simulink library "flightgear_visualization_lib"  (R2018b)
settings: Solver=VariableStepAuto  StartTime=0.0  StopTime=10.0  RelTol=1e-3
undefined symbols (not defined in the file or in its folder): fg, pos_ref
libraries: etargetslib x59, axes_transformation_lib x3, $bdroot x3, dspnetwork x2
settings Model: Creator=fabian  LastModifiedBy=yannic

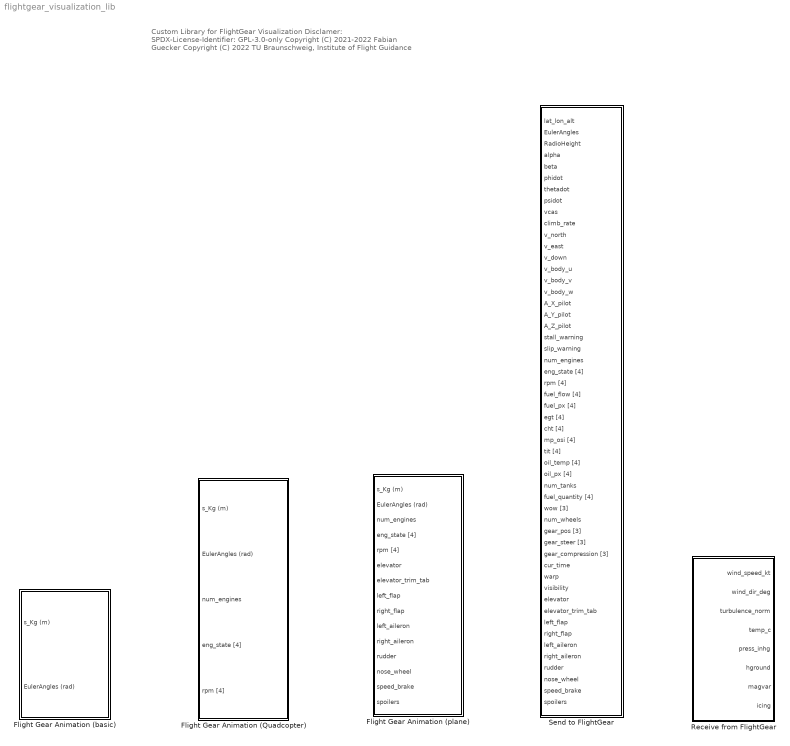
== system flightgear_visualization_lib ==
  note: Custom Library for FlightGear Visualization
      |
      | Disclamer:
      | SPDX-License-Identifier: GPL-3.0-only
      |
      | Copyright (C) 2021-2022 Fabian Guecker
      | Copyright (C) 2022 TU Braunschweig, Institute of Flight Guidance
  Flight Gear Animation (Quadcopter) : Subsystem  mask{inital_lat=pos_ref.lat, inital_long=pos_ref.lon, inital_height=pos_ref.alt, remoteURL='127.0.0.1', remotePort=5502}
      mask prompts: inital_lat "Inital Latitude (deg)"; inital_long "Inital Longitude (deg)"; inital_height "Inital Height (m)"; remoteURL "URL of FlightGear, e.g. '127.0.0.1'"; remotePort "Port of FlightGear, e.g. 5502"
      mask TypeOptions remoteURL: Send to FlightGear/remoteURL
      mask TypeOptions remotePort: Send to FlightGear/remotePort
      mask DialogControl GroupDesc Prompt: Initial Latitude
  Flight Gear Animation (basic) : Subsystem  mask{inital_lat=pos_ref.lat, inital_long=pos_ref.lon, inital_height=pos_ref.alt, remoteURL='127.0.0.1', remotePort=5502}
      mask prompts: inital_lat "Inital Latitude (deg)"; inital_long "Inital Longitude (deg)"; inital_height "Inital Height (m)"; remoteURL "URL of FlightGear, e.g. '127.0.0.1'"; remotePort "Port of FlightGear, e.g. 5502"
      mask TypeOptions remoteURL: Send to FlightGear/remoteURL
      mask TypeOptions remotePort: Send to FlightGear/remotePort
      mask DialogControl GroupDesc Prompt: Initial Latitude
  Flight Gear Animation (plane) : Subsystem  mask{inital_lat=pos_ref.lat, inital_long=pos_ref.lon, inital_height=pos_ref.alt, remoteURL='127.0.0.1', remotePort=5502}
      mask prompts: inital_lat "Inital Latitude (deg)"; inital_long "Inital Longitude (deg)"; inital_height "Inital Height (m)"; remoteURL "URL of FlightGear, e.g. '127.0.0.1'"; remotePort "Port of FlightGear, e.g. 5502"
      mask TypeOptions remoteURL: Send to FlightGear/remoteURL
      mask TypeOptions remotePort: Send to FlightGear/remotePort
      mask DialogControl GroupDesc Prompt: Initial Latitude
  Receive from FlightGear : Subsystem  mask{ip_address='127.0.0.1', ip_port=5503, sample_time=1/30, blocking_time=0, is_aerocntrl=off, is_engine=off, is_fuel=off, is_land=off, is_avionics=off, is_envir=on}
      mask prompts: ip_address "FlightGear IP address:"; ip_port "FlightGear IP port"; sample_time "Sample time, s"; blocking_time "Blocking time, s"; is_aerocntrl "Enable control surface outputs"; is_engine "Enable engine outputs"; is_fuel "Enable fuel outputs"; is_land "Enable landing outputs"; is_avionics "Enable avionics outputs"; is_envir "Enable environment outputs"
      mask init:
      | [msg_len,fg_dims,fg_type] = flightgearRcvBlockInit(is_aerocntrl,is_engine,is_fuel,...
      |     is_land,is_avionics,is_envir);
      mask DialogControl DescGroupVar Prompt: Receive from FlightGear
      mask DialogControl DescTextVar Prompt: Receive network output of FlightGear Flight Simulator.
  Send to FlightGear : Subsystem  mask{remoteURL=fg.remoteURL, remotePort=fg.remotePort}
      mask prompts: remoteURL "URL of FlightGear, e.g. 127.0.0.1"; remotePort "Port of FlightGear, e.g. 5502"

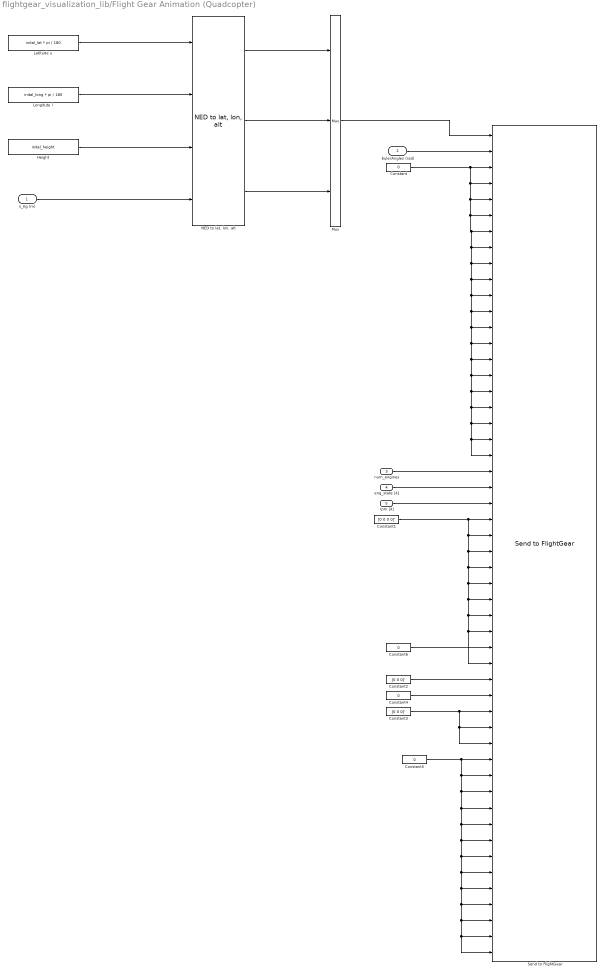
== system flightgear_visualization_lib/Flight Gear Animation (Quadcopter) ==
  s_Kg (m) : Inport
  EulerAngles (rad) : Inport  Port=2
  num_engines : Inport  Port=3  PortDimensions=[1]
  eng_state [4] : Inport  Port=4  PortDimensions=[4]
  rpm [4] : Inport  Port=5  PortDimensions=[4]
  Constant{,4..6} (4 alike) : Constant  Value=0
  Constant1 : Constant  Value=[0 0 0 0]'  VectorParams1D=off
  Constant2 : Constant  Value=[0 0 0]'  VectorParams1D=off
  Constant3 : Constant  Value=[0 0 0]'  VectorParams1D=off
  Height : Constant  Value=inital_height
  Latitude u : Constant  Value=inital_lat * pi / 180
  Longitute l : Constant  Value=inital_long * pi / 180
  Mux : Mux  Inputs=3
  "NED to lat, lon, alt" : axes_transformation_lib/NED to lat, lon, alt  SystemSampleTime=-1
      settings: SourceProductName=LADAC
  Send to FlightGear : $bdroot/Send to FlightGear  remoteURL=remoteURL  remotePort=remotePort
  wires:
  Mux/1 -> Send to FlightGear/1
  "NED to lat, lon, alt"/1 -> Mux/1
  "NED to lat, lon, alt"/2 -> Mux/2
  "NED to lat, lon, alt"/3 -> Mux/3
  Height/1 -> "NED to lat, lon, alt"/3
  Longitute l/1 -> "NED to lat, lon, alt"/2
  Latitude u/1 -> "NED to lat, lon, alt"/1
  EulerAngles (rad)/1 -> Send to FlightGear/2
  s_Kg (m)/1 -> "NED to lat, lon, alt"/4
  num_engines/1 -> Send to FlightGear/22
  eng_state [4]/1 -> Send to FlightGear/23
  rpm [4]/1 -> Send to FlightGear/24
  Constant/1 -> Send to FlightGear/3, Send to FlightGear/4, Send to FlightGear/5, Send to FlightGear/6, Send to FlightGear/7, Send to FlightGear/8, Send to FlightGear/9, Send to FlightGear/10, Send to FlightGear/11, Send to FlightGear/12, Send to FlightGear/13, Send to FlightGear/14, Send to FlightGear/15, Send to FlightGear/16, Send to FlightGear/17, Send to FlightGear/18, Send to FlightGear/19, Send to FlightGear/21, Send to FlightGear/20
  Constant1/1 -> Send to FlightGear/25, Send to FlightGear/26, Send to FlightGear/27, Send to FlightGear/28, Send to FlightGear/29, Send to FlightGear/30, Send to FlightGear/31, Send to FlightGear/32, Send to FlightGear/34
  Constant2/1 -> Send to FlightGear/35
  Constant3/1 -> Send to FlightGear/37, Send to FlightGear/39, Send to FlightGear/38
  Constant4/1 -> Send to FlightGear/36
  Constant5/1 -> Send to FlightGear/40, Send to FlightGear/41, Send to FlightGear/42, Send to FlightGear/43, Send to FlightGear/44, Send to FlightGear/45, Send to FlightGear/46, Send to FlightGear/47, Send to FlightGear/48, Send to FlightGear/49, Send to FlightGear/50, Send to FlightGear/52, Send to FlightGear/51
  Constant6/1 -> Send to FlightGear/33

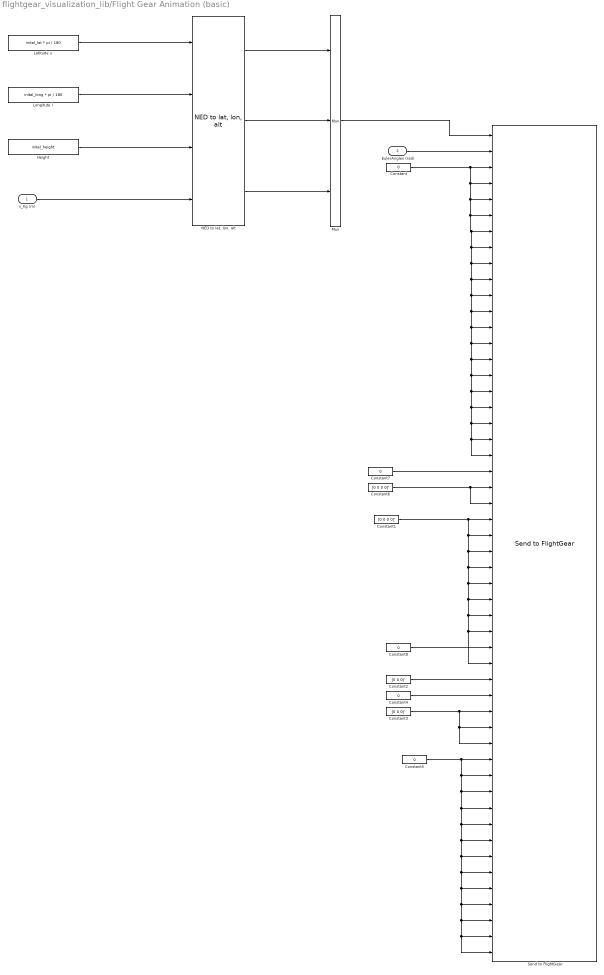
== system flightgear_visualization_lib/Flight Gear Animation (basic) ==
  s_Kg (m) : Inport
  EulerAngles (rad) : Inport  Port=2
  Constant{,4..5,8} (4 alike) : Constant  Value=0
  Constant1 : Constant  Value=[0 0 0 0]'  VectorParams1D=off
  Constant2 : Constant  Value=[0 0 0]'  VectorParams1D=off
  Constant3 : Constant  Value=[0 0 0]'  VectorParams1D=off
  Constant6 : Constant  Value=[0 0 0 0]'  VectorParams1D=off
  Constant7 : Constant  Value=0  VectorParams1D=off
  Height : Constant  Value=inital_height
  Latitude u : Constant  Value=inital_lat * pi / 180
  Longitute l : Constant  Value=inital_long * pi / 180
  Mux : Mux  Inputs=3
  "NED to lat, lon, alt" : axes_transformation_lib/NED to lat, lon, alt  SystemSampleTime=-1
      settings: SourceProductName=LADAC
  Send to FlightGear : $bdroot/Send to FlightGear  remoteURL=remoteURL  remotePort=remotePort
  wires:
  Mux/1 -> Send to FlightGear/1
  "NED to lat, lon, alt"/1 -> Mux/1
  "NED to lat, lon, alt"/2 -> Mux/2
  "NED to lat, lon, alt"/3 -> Mux/3
  Height/1 -> "NED to lat, lon, alt"/3
  Longitute l/1 -> "NED to lat, lon, alt"/2
  Latitude u/1 -> "NED to lat, lon, alt"/1
  EulerAngles (rad)/1 -> Send to FlightGear/2
  s_Kg (m)/1 -> "NED to lat, lon, alt"/4
  Constant7/1 -> Send to FlightGear/22
  Constant6/1 -> Send to FlightGear/24, Send to FlightGear/23
  Constant/1 -> Send to FlightGear/3, Send to FlightGear/4, Send to FlightGear/5, Send to FlightGear/6, Send to FlightGear/7, Send to FlightGear/8, Send to FlightGear/9, Send to FlightGear/10, Send to FlightGear/11, Send to FlightGear/12, Send to FlightGear/13, Send to FlightGear/14, Send to FlightGear/15, Send to FlightGear/16, Send to FlightGear/17, Send to FlightGear/18, Send to FlightGear/19, Send to FlightGear/21, Send to FlightGear/20
  Constant1/1 -> Send to FlightGear/25, Send to FlightGear/26, Send to FlightGear/27, Send to FlightGear/28, Send to FlightGear/29, Send to FlightGear/30, Send to FlightGear/31, Send to FlightGear/32, Send to FlightGear/34
  Constant2/1 -> Send to FlightGear/35
  Constant3/1 -> Send to FlightGear/37, Send to FlightGear/39, Send to FlightGear/38
  Constant4/1 -> Send to FlightGear/36
  Constant5/1 -> Send to FlightGear/40, Send to FlightGear/41, Send to FlightGear/42, Send to FlightGear/43, Send to FlightGear/44, Send to FlightGear/45, Send to FlightGear/46, Send to FlightGear/47, Send to FlightGear/48, Send to FlightGear/49, Send to FlightGear/50, Send to FlightGear/52, Send to FlightGear/51
  Constant8/1 -> Send to FlightGear/33

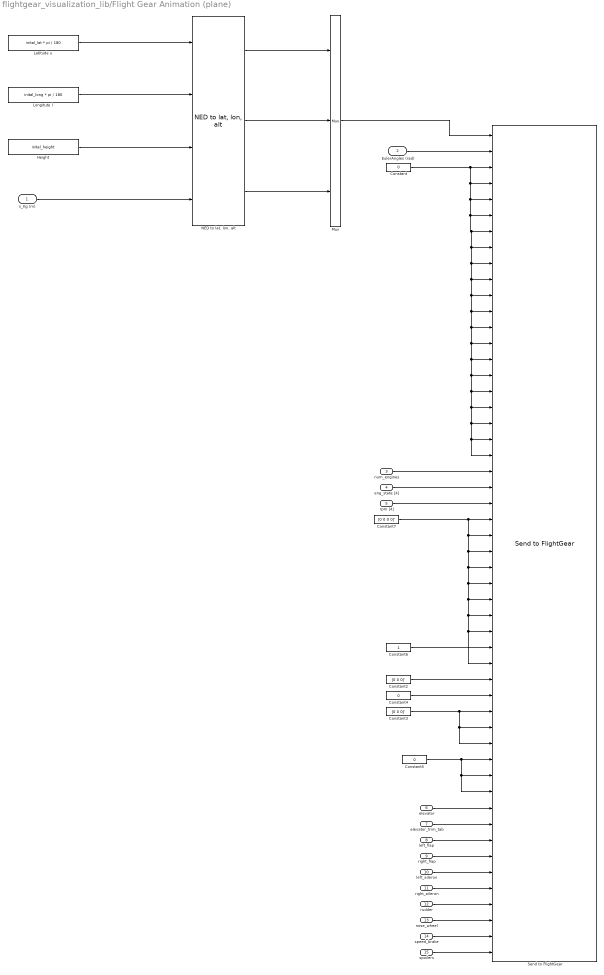
== system flightgear_visualization_lib/Flight Gear Animation (plane) ==
  s_Kg (m) : Inport
  EulerAngles (rad) : Inport  Port=2
  num_engines : Inport  Port=3  PortDimensions=[1]
  eng_state [4] : Inport  Port=4  PortDimensions=[4]
  rpm [4] : Inport  Port=5  PortDimensions=[4]
  elevator : Inport  Port=6  PortDimensions=[1]
  elevator_trim_tab : Inport  Port=7  PortDimensions=[1]
  left_flap : Inport  Port=8  PortDimensions=[1]
  right_flap : Inport  Port=9  PortDimensions=[1]
  left_aileron : Inport  Port=10  PortDimensions=[1]
  right_aileron : Inport  Port=11  PortDimensions=[1]
  rudder : Inport  Port=12  PortDimensions=[1]
  nose_wheel : Inport  Port=13  PortDimensions=[1]
  speed_brake : Inport  Port=14  PortDimensions=[1]
  spoilers : Inport  Port=15  PortDimensions=[1]
  Constant : Constant  Value=0
  Constant2 : Constant  Value=[0 0 0]'  VectorParams1D=off
  Constant3 : Constant  Value=[0 0 0]'  VectorParams1D=off
  Constant4 : Constant  Value=0
  Constant5 : Constant  Value=0
  Constant6 : Constant
  Constant7 : Constant  Value=[0 0 0 0]'  VectorParams1D=off
  Height : Constant  Value=inital_height
  Latitude u : Constant  Value=inital_lat * pi / 180
  Longitute l : Constant  Value=inital_long * pi / 180
  Mux : Mux  Inputs=3
  "NED to lat, lon, alt" : axes_transformation_lib/NED to lat, lon, alt  SystemSampleTime=-1
      settings: SourceProductName=LADAC
  Send to FlightGear : $bdroot/Send to FlightGear  remoteURL=remoteURL  remotePort=remotePort
  wires:
  Mux/1 -> Send to FlightGear/1
  "NED to lat, lon, alt"/1 -> Mux/1
  "NED to lat, lon, alt"/2 -> Mux/2
  "NED to lat, lon, alt"/3 -> Mux/3
  Height/1 -> "NED to lat, lon, alt"/3
  Longitute l/1 -> "NED to lat, lon, alt"/2
  Latitude u/1 -> "NED to lat, lon, alt"/1
  EulerAngles (rad)/1 -> Send to FlightGear/2
  s_Kg (m)/1 -> "NED to lat, lon, alt"/4
  spoilers/1 -> Send to FlightGear/52
  speed_brake/1 -> Send to FlightGear/51
  nose_wheel/1 -> Send to FlightGear/50
  rudder/1 -> Send to FlightGear/49
  elevator/1 -> Send to FlightGear/43
  elevator_trim_tab/1 -> Send to FlightGear/44
  left_flap/1 -> Send to FlightGear/45
  right_flap/1 -> Send to FlightGear/46
  left_aileron/1 -> Send to FlightGear/47
  right_aileron/1 -> Send to FlightGear/48
  num_engines/1 -> Send to FlightGear/22
  eng_state [4]/1 -> Send to FlightGear/23
  rpm [4]/1 -> Send to FlightGear/24
  Constant/1 -> Send to FlightGear/3, Send to FlightGear/4, Send to FlightGear/5, Send to FlightGear/6, Send to FlightGear/7, Send to FlightGear/8, Send to FlightGear/9, Send to FlightGear/10, Send to FlightGear/11, Send to FlightGear/12, Send to FlightGear/13, Send to FlightGear/14, Send to FlightGear/15, Send to FlightGear/16, Send to FlightGear/17, Send to FlightGear/18, Send to FlightGear/19, Send to FlightGear/21, Send to FlightGear/20
  Constant7/1 -> Send to FlightGear/25, Send to FlightGear/26, Send to FlightGear/27, Send to FlightGear/28, Send to FlightGear/29, Send to FlightGear/30, Send to FlightGear/31, Send to FlightGear/32, Send to FlightGear/34
  Constant2/1 -> Send to FlightGear/35
  Constant3/1 -> Send to FlightGear/37, Send to FlightGear/39, Send to FlightGear/38
  Constant4/1 -> Send to FlightGear/36
  Constant5/1 -> Send to FlightGear/40, Send to FlightGear/42, Send to FlightGear/41
  Constant6/1 -> Send to FlightGear/33

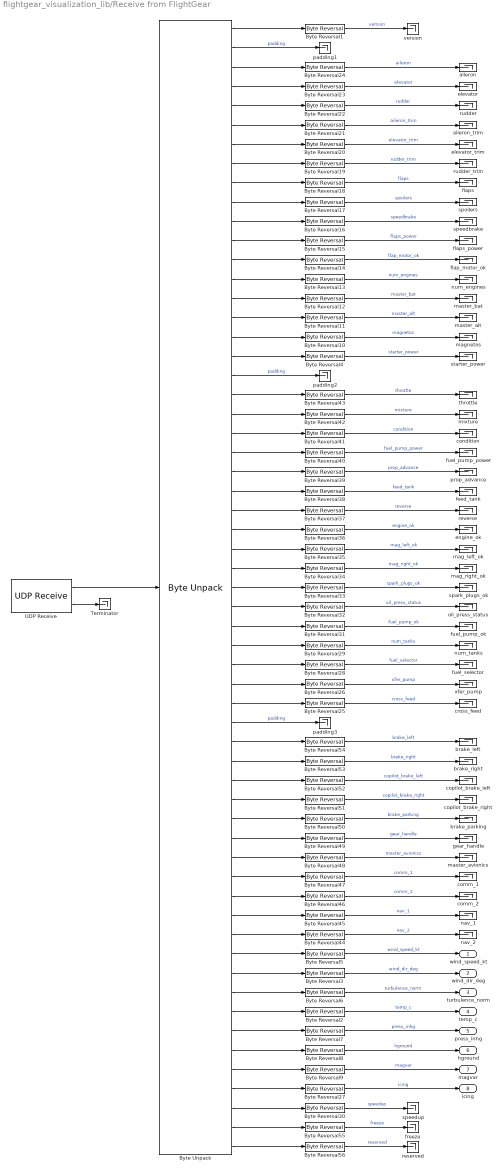
== system flightgear_visualization_lib/Receive from FlightGear ==
  Byte Reversal{1..56} (56 alike) : etargetslib/Byte Reversal  numInp=1
  Byte Unpack : etargetslib/Byte Unpack  dimensions=fg_dims  datatypes=fg_type  byteAlign=1
  Terminator : Terminator
  UDP Receive : dspnetwork/UDP Receive  localURL='0.0.0.0'  localPort=ip_port  remoteURL=ip_address  remotePort=-1  recvBufferSize=msg_len  dims=msg_len  signalDatatype=uint8  isVarSize=off  showBlockingTime=on  blockingTime=blocking_time  sampletime=sample_time  blockPlatform=HOST
      settings: SourceProductName=DSP System Toolbox  SourceProductBaseCode=DS
  aileron : Terminator
  aileron_trim : Terminator
  brake_left : Terminator
  brake_parking : Terminator
  brake_right : Terminator
  comm_1 : Terminator
  comm_2 : Terminator
  condition : Terminator
  copilot_brake_left : Terminator
  copilot_brake_right : Terminator
  cross_feed : Terminator
  elevator : Terminator
  elevator_trim : Terminator
  engine_ok : Terminator
  feed_tank : Terminator
  flap_motor_ok : Terminator
  flaps : Terminator
  flaps_power : Terminator
  freeze : Terminator
  fuel_pump_ok : Terminator
  fuel_pump_power : Terminator
  fuel_selector : Terminator
  gear_handle : Terminator
  mag_left_ok : Terminator
  mag_right_ok : Terminator
  magnetos : Terminator
  master_alt : Terminator
  master_avionics : Terminator
  master_bat : Terminator
  mixture : Terminator
  nav_1 : Terminator
  nav_2 : Terminator
  num_engines : Terminator
  num_tanks : Terminator
  oil_press_status : Terminator
  padding1 : Terminator
  padding2 : Terminator
  padding3 : Terminator
  prop_advance : Terminator
  reserved : Terminator
  reverse : Terminator
  rudder : Terminator
  rudder_trim : Terminator
  spark_plugs_ok : Terminator
  speedbrake : Terminator
  speedup : Terminator
  spoilers : Terminator
  starter_power : Terminator
  throttle : Terminator
  version : Terminator
  xfer_pump : Terminator
  wind_speed_kt : Outport
  wind_dir_deg : Outport  Port=2
  turbulence_norm : Outport  Port=3
  temp_c : Outport  Port=4
  press_inhg : Outport  Port=5
  hground : Outport  Port=6
  magvar : Outport  Port=7
  icing : Outport  Port=8
  wires:
  Byte Unpack/23 -> Byte Reversal40/1
  Byte Reversal46/1 -> comm_2/1  "comm_2"
  Byte Unpack/54 -> Byte Reversal8/1
  Byte Unpack/55 -> Byte Reversal9/1
  Byte Reversal28/1 -> fuel_selector/1  "fuel_selector"
  Byte Unpack/7 -> Byte Reversal20/1
  Byte Reversal36/1 -> engine_ok/1  "engine_ok"
  Byte Unpack/57 -> Byte Reversal30/1
  Byte Unpack/48 -> Byte Reversal44/1
  Byte Reversal11/1 -> master_alt/1  "master_alt"
  UDP Receive/1 -> Byte Unpack/1
  Byte Unpack/36 -> Byte Reversal25/1
  Byte Unpack/19 -> padding2/1  "padding"
  Byte Reversal12/1 -> master_bat/1  "master_bat"
  Byte Unpack/10 -> Byte Reversal17/1
  Byte Unpack/17 -> Byte Reversal10/1
  Byte Reversal16/1 -> speedbrake/1  "speedbrake"
  Byte Reversal7/1 -> press_inhg/1  "press_inhg"
  Byte Reversal54/1 -> brake_left/1  "brake_left"
  Byte Unpack/1 -> Byte Reversal1/1
  Byte Reversal49/1 -> gear_handle/1  "gear_handle"
  Byte Unpack/15 -> Byte Reversal12/1
  Byte Reversal24/1 -> aileron/1  "aileron"
  Byte Reversal10/1 -> magnetos/1  "magnetos"
  Byte Unpack/50 -> Byte Reversal3/1
  Byte Unpack/8 -> Byte Reversal19/1
  Byte Reversal4/1 -> starter_power/1  "starter_power"
  Byte Reversal20/1 -> elevator_trim/1  "elevator_trim"
  Byte Unpack/18 -> Byte Reversal4/1
  Byte Unpack/43 -> Byte Reversal49/1
  Byte Unpack/41 -> Byte Reversal51/1
  Byte Unpack/44 -> Byte Reversal48/1
  Byte Unpack/6 -> Byte Reversal21/1
  Byte Unpack/59 -> Byte Reversal56/1
  Byte Unpack/35 -> Byte Reversal26/1
  Byte Unpack/49 -> Byte Reversal5/1
  Byte Unpack/38 -> Byte Reversal54/1
  Byte Reversal31/1 -> fuel_pump_ok/1  "fuel_pump_ok"
  Byte Reversal5/1 -> wind_speed_kt/1  "wind_speed_kt"
  Byte Reversal18/1 -> flaps/1  "flaps"
  Byte Unpack/5 -> Byte Reversal22/1
  Byte Reversal41/1 -> condition/1  "condition"
  Byte Reversal22/1 -> rudder/1  "rudder"
  Byte Unpack/45 -> Byte Reversal47/1
  Byte Unpack/46 -> Byte Reversal46/1
  Byte Unpack/25 -> Byte Reversal38/1
  Byte Reversal42/1 -> mixture/1  "mixture"
  UDP Receive/2 -> Terminator/1
  Byte Reversal2/1 -> temp_c/1  "temp_c"
  Byte Unpack/26 -> Byte Reversal37/1
  Byte Reversal37/1 -> reverse/1  "reverse"
  Byte Unpack/30 -> Byte Reversal33/1
  Byte Unpack/47 -> Byte Reversal45/1
  Byte Unpack/58 -> Byte Reversal55/1
  Byte Unpack/33 -> Byte Reversal29/1
  Byte Reversal34/1 -> mag_right_ok/1  "mag_right_ok"
  Byte Unpack/39 -> Byte Reversal53/1
  Byte Reversal9/1 -> magvar/1  "magvar"
  Byte Reversal17/1 -> spoilers/1  "spoilers"
  Byte Reversal6/1 -> turbulence_norm/1  "turbulence_norm"
  Byte Reversal47/1 -> comm_1/1  "comm_1"
  Byte Unpack/9 -> Byte Reversal18/1
  Byte Unpack/53 -> Byte Reversal7/1
  Byte Unpack/37 -> padding3/1  "padding"
  Byte Reversal48/1 -> master_avionics/1  "master_avionics"
  Byte Unpack/22 -> Byte Reversal41/1
  Byte Unpack/28 -> Byte Reversal35/1
  Byte Reversal44/1 -> nav_2/1  "nav_2"
  Byte Unpack/20 -> Byte Reversal43/1
  Byte Reversal13/1 -> num_engines/1  "num_engines"
  Byte Reversal27/1 -> icing/1  "icing"
  Byte Reversal3/1 -> wind_dir_deg/1  "wind_dir_deg"
  Byte Unpack/42 -> Byte Reversal50/1
  Byte Unpack/34 -> Byte Reversal28/1
  Byte Reversal8/1 -> hground/1  "hground"
  Byte Reversal14/1 -> flap_motor_ok/1  "flap_motor_ok"
  Byte Reversal33/1 -> spark_plugs_ok/1  "spark_plugs_ok"
  Byte Unpack/12 -> Byte Reversal15/1
  Byte Unpack/16 -> Byte Reversal11/1
  Byte Unpack/13 -> Byte Reversal14/1
  Byte Reversal32/1 -> oil_press_status/1  "oil_press_status"
  Byte Reversal29/1 -> num_tanks/1  "num_tanks"
  Byte Reversal43/1 -> throttle/1  "throttle"
  Byte Reversal21/1 -> aileron_trim/1  "aileron_trim"
  Byte Reversal30/1 -> speedup/1  "speedup"
  Byte Reversal40/1 -> fuel_pump_power/1  "fuel_pump_power"
  Byte Reversal50/1 -> brake_parking/1  "brake_parking"
  Byte Reversal52/1 -> copilot_brake_left/1  "copilot_brake_left"
  Byte Unpack/40 -> Byte Reversal52/1
  Byte Unpack/11 -> Byte Reversal16/1
  Byte Reversal53/1 -> brake_right/1  "brake_right"
  Byte Reversal45/1 -> nav_1/1  "nav_1"
  Byte Unpack/14 -> Byte Reversal13/1
  Byte Reversal56/1 -> reserved/1  "reserved"
  Byte Unpack/2 -> padding1/1  "padding"
  Byte Reversal15/1 -> flaps_power/1  "flaps_power"
  Byte Unpack/31 -> Byte Reversal32/1
  Byte Unpack/24 -> Byte Reversal39/1
  Byte Reversal51/1 -> copilot_brake_right/1  "copilot_brake_right"
  Byte Reversal25/1 -> cross_feed/1  "cross_feed"
  Byte Unpack/32 -> Byte Reversal31/1
  Byte Reversal1/1 -> version/1  "version"
  Byte Unpack/51 -> Byte Reversal6/1
  Byte Reversal38/1 -> feed_tank/1  "feed_tank"
  Byte Reversal39/1 -> prop_advance/1  "prop_advance"
  Byte Reversal26/1 -> xfer_pump/1  "xfer_pump"
  Byte Unpack/56 -> Byte Reversal27/1
  Byte Reversal35/1 -> mag_left_ok/1  "mag_left_ok"
  Byte Reversal19/1 -> rudder_trim/1  "rudder_trim"
  Byte Unpack/29 -> Byte Reversal34/1
  Byte Unpack/52 -> Byte Reversal2/1
  Byte Unpack/21 -> Byte Reversal42/1
  Byte Unpack/3 -> Byte Reversal24/1
  Byte Reversal55/1 -> freeze/1  "freeze"
  Byte Reversal23/1 -> elevator/1  "elevator"
  Byte Unpack/27 -> Byte Reversal36/1
  Byte Unpack/4 -> Byte Reversal23/1

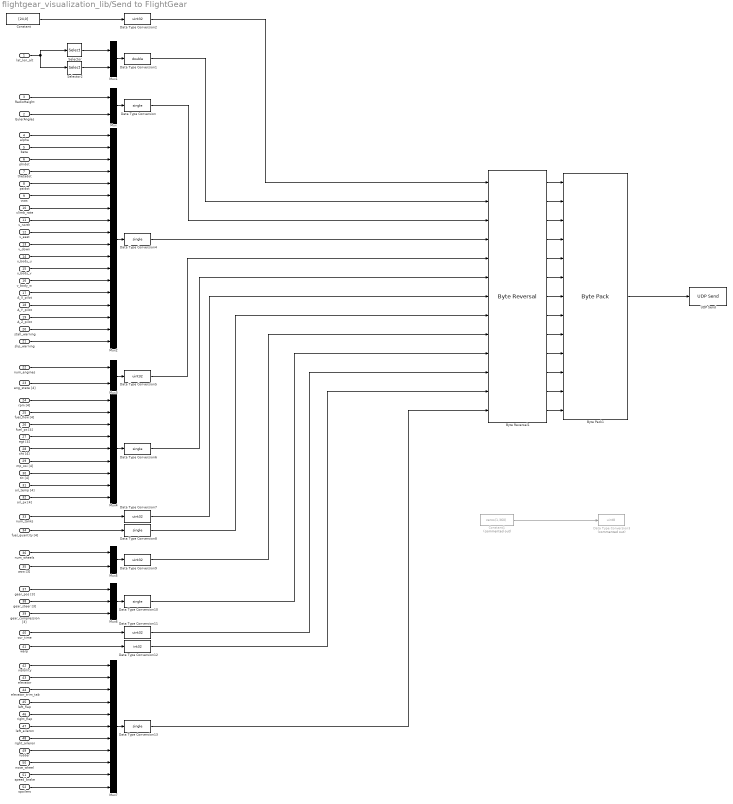
== system flightgear_visualization_lib/Send to FlightGear ==
  lat_lon_alt : Inport  PortDimensions=[3]
  EulerAngles : Inport  Port=2  PortDimensions=[3]
  RadioHeight : Inport  Port=3  PortDimensions=[1]
  alpha : Inport  Port=4  PortDimensions=[1]
  beta : Inport  Port=5  PortDimensions=[1]
  phidot : Inport  Port=6  PortDimensions=[1]
  thetadot : Inport  Port=7  PortDimensions=[1]
  psidot : Inport  Port=8  PortDimensions=[1]
  vcas : Inport  Port=9  PortDimensions=[1]
  climb_rate : Inport  Port=10  PortDimensions=[1]
  v_north : Inport  Port=11  PortDimensions=[1]
  v_east : Inport  Port=12  PortDimensions=[1]
  v_down : Inport  Port=13  PortDimensions=[1]
  v_body_u : Inport  Port=14  PortDimensions=[1]
  v_body_v : Inport  Port=15  PortDimensions=[1]
  v_body_w : Inport  Port=16  PortDimensions=[1]
  A_X_pilot : Inport  Port=17  PortDimensions=[1]
  A_Y_pilot : Inport  Port=18  PortDimensions=[1]
  A_Z_pilot : Inport  Port=19  PortDimensions=[1]
  stall_warning : Inport  Port=20  PortDimensions=[1]
  slip_warning : Inport  Port=21  PortDimensions=[1]
  num_engines : Inport  Port=22  PortDimensions=[1]
  eng_state [4] : Inport  Port=23  PortDimensions=[4]
  rpm [4] : Inport  Port=24  PortDimensions=[4]
  fuel_flow [4] : Inport  Port=25  PortDimensions=[4]
  fuel_px [4] : Inport  Port=26  PortDimensions=[4]
  egt [4] : Inport  Port=27  PortDimensions=[4]
  cht [4] : Inport  Port=28  PortDimensions=[4]
  mp_osi [4] : Inport  Port=29  PortDimensions=[4]
  tit [4] : Inport  Port=30  PortDimensions=[4]
  oil_temp [4] : Inport  Port=31  PortDimensions=[4]
  oil_px [4] : Inport  Port=32  PortDimensions=[4]
  num_tanks : Inport  Port=33  PortDimensions=[1]
  fuel_quantity [4] : Inport  Port=34  PortDimensions=[4]
  wow [3] : Inport  Port=35  PortDimensions=[3]
  num_wheels : Inport  Port=36  PortDimensions=[1]
  gear_pos [3] : Inport  Port=37  PortDimensions=[3]
  gear_steer [3] : Inport  Port=38  PortDimensions=[3]
  gear_compression [3] : Inport  Port=39  PortDimensions=[3]
  cur_time : Inport  Port=40  PortDimensions=[1]
  warp : Inport  Port=41  PortDimensions=[1]
  visibility : Inport  Port=42  PortDimensions=[1]
  elevator : Inport  Port=43  PortDimensions=[1]
  elevator_trim_tab : Inport  Port=44  PortDimensions=[1]
  left_flap : Inport  Port=45  PortDimensions=[1]
  right_flap : Inport  Port=46  PortDimensions=[1]
  left_aileron : Inport  Port=47  PortDimensions=[1]
  right_aileron : Inport  Port=48  PortDimensions=[1]
  rudder : Inport  Port=49  PortDimensions=[1]
  nose_wheel : Inport  Port=50  PortDimensions=[1]
  speed_brake : Inport  Port=51  PortDimensions=[1]
  spoilers : Inport  Port=52  PortDimensions=[1]
  Byte Pack1 : etargetslib/Byte Pack  datatypes={'uint32','double','single','single','uint32','single','uint32','single','uint32','single','uint32','int32','single'}  byteAlign=1
  Byte Reversal1 : etargetslib/Byte Reversal  numInp=13
  Constant : Constant  Value=[24,0]
  Constant1 : Constant  Commented=on  Value=zeros(1,360)
  Data Type Conversion{,4,6,8,10,13} (6 alike) : DataTypeConversion  OutDataTypeStr=single
  Data Type Conversion1 : DataTypeConversion  OutDataTypeStr=double
  Data Type Conversion{2,5,7,9,11} (5 alike) : DataTypeConversion  OutDataTypeStr=uint32
  Data Type Conversion12 : DataTypeConversion  OutDataTypeStr=int32
  Data Type Conversion3 : DataTypeConversion  Commented=on  OutDataTypeStr=uint8
  Mux{,1,3,5} (4 alike) : Mux  Inputs=2
  Mux2 : Mux  Inputs=18
  Mux4 : Mux  Inputs=9
  Mux6 : Mux  Inputs=3
  Mux7 : Mux  Inputs=11
  Selector : Selector  InputPortWidth=3  IndexOptions=Index vector (dialog)  Indices=[2 1]  OutputSizes=1
  Selector2 : Selector  InputPortWidth=3  IndexOptions=Index vector (dialog)  Indices=[3]  OutputSizes=1
  UDP Send : dspnetwork/UDP Send  remoteURL=remoteURL  remotePort=remotePort  localURL='0.0.0.0'  localPortSource=Automatically determine  localPort=-1  sampletime=-1  blockPlatform=[]  separateLengthPort=0
      settings: SourceProductName=DSP System Toolbox  SourceProductBaseCode=DS
  wires:
  Byte Pack1/1 -> UDP Send/1
  Byte Reversal1/2 -> Byte Pack1/2
  Byte Reversal1/3 -> Byte Pack1/3
  Byte Reversal1/1 -> Byte Pack1/1
  Constant/1 -> Data Type Conversion2/1
  Data Type Conversion2/1 -> Byte Reversal1/1
  Data Type Conversion1/1 -> Byte Reversal1/2
  Byte Reversal1/4 -> Byte Pack1/4
  Constant1/1 -> Data Type Conversion3/1
  EulerAngles/1 -> Mux/2
  RadioHeight/1 -> Mux/1
  Mux/1 -> Data Type Conversion/1
  Mux1/1 -> Data Type Conversion1/1
  Data Type Conversion/1 -> Byte Reversal1/3
  Selector/1 -> Mux1/1
  lat_lon_alt/1 -> Selector2/1, Selector/1
  Selector2/1 -> Mux1/2
  Byte Reversal1/5 -> Byte Pack1/5
  Mux2/1 -> Data Type Conversion4/1
  alpha/1 -> Mux2/1
  beta/1 -> Mux2/2
  phidot/1 -> Mux2/3
  thetadot/1 -> Mux2/4
  psidot/1 -> Mux2/5
  vcas/1 -> Mux2/6
  climb_rate/1 -> Mux2/7
  v_north/1 -> Mux2/8
  v_east/1 -> Mux2/9
  v_down/1 -> Mux2/10
  v_body_u/1 -> Mux2/11
  v_body_v/1 -> Mux2/12
  v_body_w/1 -> Mux2/13
  A_X_pilot/1 -> Mux2/14
  A_Y_pilot/1 -> Mux2/15
  A_Z_pilot/1 -> Mux2/16
  stall_warning/1 -> Mux2/17
  slip_warning/1 -> Mux2/18
  Data Type Conversion4/1 -> Byte Reversal1/4
  Mux3/1 -> Data Type Conversion5/1
  Data Type Conversion5/1 -> Byte Reversal1/5
  mp_osi [4]/1 -> Mux4/6
  fuel_flow [4]/1 -> Mux4/2
  egt [4]/1 -> Mux4/4
  cht [4]/1 -> Mux4/5
  rpm [4]/1 -> Mux4/1
  fuel_px [4]/1 -> Mux4/3
  Mux4/1 -> Data Type Conversion6/1
  Data Type Conversion6/1 -> Byte Reversal1/6
  Byte Reversal1/6 -> Byte Pack1/6
  oil_temp [4]/1 -> Mux4/8
  oil_px [4]/1 -> Mux4/9
  tit [4]/1 -> Mux4/7
  num_tanks/1 -> Data Type Conversion7/1
  fuel_quantity [4]/1 -> Data Type Conversion8/1
  wow [3]/1 -> Mux5/2
  num_wheels/1 -> Mux5/1
  Mux5/1 -> Data Type Conversion9/1
  gear_pos [3]/1 -> Mux6/1
  gear_compression [3]/1 -> Mux6/3
  gear_steer [3]/1 -> Mux6/2
  Mux6/1 -> Data Type Conversion10/1
  cur_time/1 -> Data Type Conversion11/1
  warp/1 -> Data Type Conversion12/1
  nose_wheel/1 -> Mux7/9
  left_flap/1 -> Mux7/4
  right_aileron/1 -> Mux7/7
  elevator/1 -> Mux7/2
  Mux7/1 -> Data Type Conversion13/1
  elevator_trim_tab/1 -> Mux7/3
  left_aileron/1 -> Mux7/6
  right_flap/1 -> Mux7/5
  visibility/1 -> Mux7/1
  rudder/1 -> Mux7/8
  spoilers/1 -> Mux7/11
  speed_brake/1 -> Mux7/10
  Data Type Conversion7/1 -> Byte Reversal1/7
  Data Type Conversion8/1 -> Byte Reversal1/8
  Byte Reversal1/7 -> Byte Pack1/7
  Byte Reversal1/8 -> Byte Pack1/8
  Byte Reversal1/9 -> Byte Pack1/9
  Byte Reversal1/10 -> Byte Pack1/10
  Byte Reversal1/11 -> Byte Pack1/11
  Byte Reversal1/12 -> Byte Pack1/12
  Byte Reversal1/13 -> Byte Pack1/13
  Data Type Conversion9/1 -> Byte Reversal1/9
  Data Type Conversion10/1 -> Byte Reversal1/10
  Data Type Conversion11/1 -> Byte Reversal1/11
  Data Type Conversion12/1 -> Byte Reversal1/12
  Data Type Conversion13/1 -> Byte Reversal1/13
  num_engines/1 -> Mux3/1
  eng_state [4]/1 -> Mux3/2
